simulink model "RLS_ADRC_2nd_order_Kang"  (R2024b)
settings: Solver=FixedStepAuto  StartTime=0.0  StopTime=250  FixedStep=T_sample  RelTol=1e-3
undefined symbols (not defined in the file): T_sample
settings Model: Creator=songk  LastModifiedBy=sk3547969879
settings RTWCC: GPUComputeCapability=3.5

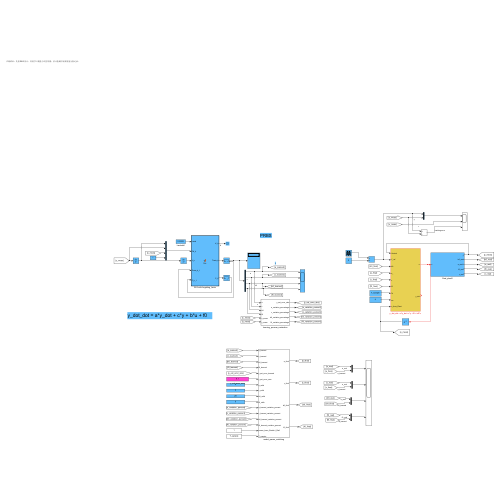
[thumbnail: Simulink's stored preview of the top-level diagram]
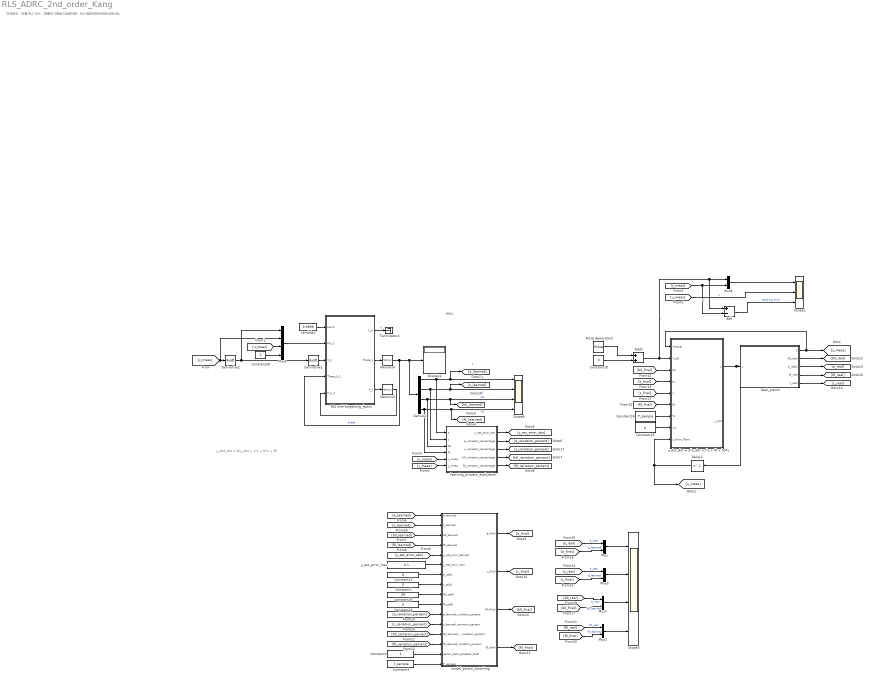
== system RLS_ADRC_2nd_order_Kang ==
  note: t
  note: PRBS
  note: y_dot_dot = a*y_dot + c*y + b*u + f0
  note: 在线辨识：先看 RLS 估计，再看学习使能与误差判据；估计值和控制采用值分别记录。
  Add : Sum  Inputs=+-
  Add2 : Sum
  Constant{1,20,22..23} (4 alike) : Constant  Value=0
  Constant2 : Constant
  Constant24 : Constant  Value=T_sample
  Constant25 : Constant  Value=4
  Constant26 : Constant  Value=28
  Constant28 : Constant
  Constant3 : Constant  Value=T_sample
  Delay2 : Delay  DelayLength=1
  Demux2 : Demux
  Derivative1 : Derivative
  Derivative2 : Derivative
  Display2 : Display
  Lambda2 : Constant  Value=0.9999
  Memory4 : Memory  InitialCondition=[1e-10;1e-10;1e-10;1e-10;]  InheritSampleTime=on
  Memory5 : Memory  InitialCondition=[1,0,0 0; 0,1,0 0; 0,0,1,0; 0 0 0 1]  InheritSampleTime=on
  Mux{,1..4} (5 alike) : Mux  Inputs=2
  Mux5 : Mux
  Pulse Generator2 : DiscretePulseGenerator  PulseType=Time based  Period=10  PulseWidth=50
  RLS with forgetting_factor : MATLAB Function  TreatAsAtomicUnit=on
  Real_plant2 : Subsystem
  Scope1 : Scope  NumInputPorts=3
  Scope3 : Scope  NumInputPorts=4
  Scope6 : Scope  NumInputPorts=4
  Terminator2 : Terminator
  learning_process_evaluation : Subsystem
  model_param_switching : Subsystem
  "y_dot_dot = a*y_dot +c*y + f0 + b0*u " : Subsystem
  y_est_error_max : Constant  Value=0.1
  wires:
  Real_plant2/1(y) -> "y_dot_dot = a*y_dot +c*y + f0 + b0*u "/1(Yactual), [y_meas]
  RLS with forgetting_factor/3(P_k) -> Memory5/1
  Derivative2/1 -> Derivative1/1, Mux5/1
  Memory4/1 -> RLS with forgetting_factor/4(Theta_k_1), Demux2/1, Display2/1  "theta"
  "y_dot_dot = a*y_dot +c*y + f0 + b0*u "/1(u) -> Delay2/1, Real_plant2/1(u)
  Mux4/1 -> Scope1/1
  RLS with forgetting_factor/2(Theta_k) -> Memory4/1
  Lambda2/1 -> RLS with forgetting_factor/1(Lamb)
  Demux2/4 -> Scope6/4, [f0_learned], learning_process_evaluation/4(f0)  "f0"
  Memory5/1 -> RLS with forgetting_factor/5(P_k_1)
  Pulse Generator2/1 -> Add2/1
  Constant28/1 -> Mux5/4
  Add2/1 -> Add/1, Mux4/1, "y_dot_dot = a*y_dot +c*y + f0 + b0*u "/2(Y_ref)  "r"
  Mux5/1 -> RLS with forgetting_factor/2(Phi_k)
  RLS with forgetting_factor/1(K_k) -> Terminator2/1  "K"
  Constant24/1 -> "y_dot_dot = a*y_dot +c*y + f0 + b0*u "/7(Ts)
  Constant20/1 -> Add2/2
  Constant25/1 -> "y_dot_dot = a*y_dot +c*y + f0 + b0*u "/8(wc)
  [y_meas] -> Mux5/2, Derivative2/1
  [u_meas] -> Mux5/3
  [y_meas] -> Add/2, Mux4/2  "y"
  [u_meas] -> Scope1/2  "u"
  Demux2/1 -> [a_learned], Scope6/1, learning_process_evaluation/1(a)  "a"
  Demux2/3 -> Scope6/3, [b0_learned], learning_process_evaluation/3(b0)  "b0"
  learning_process_evaluation/2(a_variation_percentage) -> [a_variation_percent]
  learning_process_evaluation/1(y_est_error_abs) -> [y_est_error_abs]
  learning_process_evaluation/4(b0_variation_percentage) -> [b0_variation_percent]
  learning_process_evaluation/5(f0_variation_percentage) -> [f0_variation_percent]
  [y_meas] -> learning_process_evaluation/6(y_meas)
  [u_meas] -> learning_process_evaluation/5(u_meas)
  [a_learned] -> model_param_switching/1(a_learned)
  [b0_learned] -> model_param_switching/3(b0_learned)
  [f0_learned] -> model_param_switching/4(f0_learned)
  [y_est_error_abs] -> model_param_switching/5(y_est_error_learned)
  y_est_error_max/1 -> model_param_switching/6(y_est_erorr_max)
  Constant23/1 -> model_param_switching/7(a_calib)
  Constant26/1 -> model_param_switching/9(b0_calib)
  Constant22/1 -> model_param_switching/10(f0_calib)
  [a_variation_percent] -> model_param_switching/11(a_learned_variation_percent)
  [b0_variation_percent] -> model_param_switching/13(b0_learned_variation_percent)
  model_param_switching/1(a_final) -> [a_final]
  model_param_switching/3(b0_final) -> [b0_final]
  [a_final] -> "y_dot_dot = a*y_dot +c*y + f0 + b0*u "/4(a_)
  [b0_final] -> "y_dot_dot = a*y_dot +c*y + f0 + b0*u "/3(b0)
  [f0_final] -> "y_dot_dot = a*y_dot +c*y + f0 + b0*u "/6(f0)
  Real_plant2/2(b0_real) -> [b0_real]
  Real_plant2/3(a_real1) -> [a_real]
  Real_plant2/5(c_real) -> [c_real]
  [a_real] -> Mux/1  "a_real"
  [a_final] -> Mux/2  "a_learned"
  [b0_real] -> Mux1/1  "b_real"
  [b0_final] -> Mux1/2  "b0_learned"
  [f0_real] -> Mux2/1  "f0_real"
  [f0_final] -> Mux2/2  "f0_learned"
  Mux/1 -> Scope3/1
  Mux1/1 -> Scope3/3
  Mux2/1 -> Scope3/4
  Add/1 -> Scope1/3  "tracking error"
  Real_plant2/4(f0_real) -> [f0_real]
  [c_final] -> "y_dot_dot = a*y_dot +c*y + f0 + b0*u "/5(c)
  Mux3/1 -> Scope3/2
  [c_final] -> Mux3/2  "a_learned"
  [c_real] -> Mux3/1  "a_real"
  model_param_switching/2(c_final) -> [c_final]
  model_param_switching/4(f0_final) -> [f0_final]
  Constant3/1 -> model_param_switching/16(T_sample)
  [f0_variation_percent] -> model_param_switching/14(f0_learned_variation_percent)
  [c_variation_percent] -> model_param_switching/12(c_learned_variation_percent)
  Constant1/1 -> model_param_switching/8(c_calib)
  [c_learned] -> model_param_switching/2(c_learned)
  learning_process_evaluation/3(c_variation_percentage) -> [c_variation_percent]
  Demux2/2 -> learning_process_evaluation/2(c), [c_learned], Scope6/2  "c"
  Derivative1/1 -> RLS with forgetting_factor/3(Y_k)
  Constant2/1 -> model_param_switching/15(param_learn_Enable1_Dis0)
  Delay2/1 -> "y_dot_dot = a*y_dot +c*y + f0 + b0*u "/9(u_from_Plant), [u_meas]

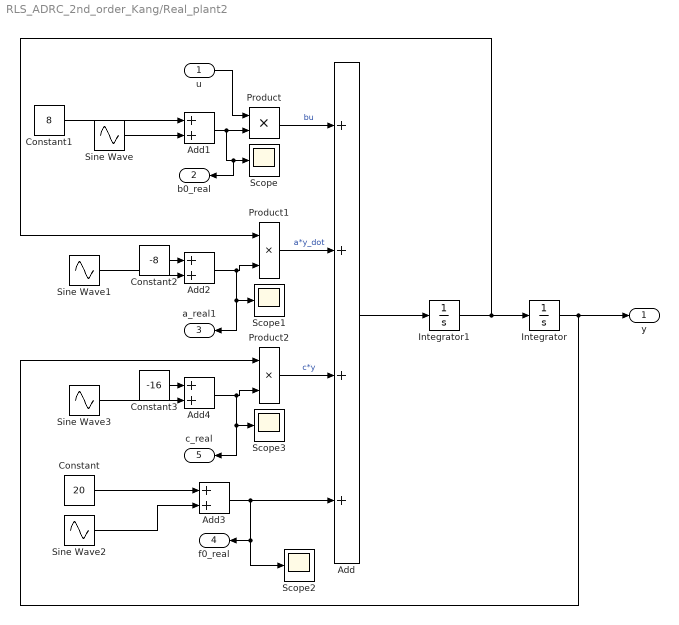
== system RLS_ADRC_2nd_order_Kang/Real_plant2 ==
  u : Inport
  Add : Sum  Inputs=++++
  Add{1..4} (4 alike) : Sum
  Constant : Constant  Value=20
  Constant1 : Constant  Value=8
  Constant2 : Constant  Value=-8
  Constant3 : Constant  Value=-16
  Integrator : Integrator
  Integrator1 : Integrator
  Product : Product
  Product1 : Product
  Product2 : Product
  Scope{,1..3} (4 alike) : Scope
  Sine Wave : Sin  Amplitude=10*0  Frequency=0.0125*2  SampleTime=0
  Sine Wave1 : Sin  Amplitude=0.2*0  Frequency=0.0125*2  Phase=90/180*pi  SampleTime=0
  Sine Wave2 : Sin  Amplitude=100*0  Frequency=0.009*3  Phase=180/180*pi  SampleTime=0
  Sine Wave3 : Sin  Amplitude=0.2*0  Frequency=0.0125*2  Phase=90/180*pi  SampleTime=0
  y : Outport
  b0_real : Outport  Port=2
  a_real1 : Outport  Port=3
  f0_real : Outport  Port=4
  c_real : Outport  Port=5
  wires:
  Add/1 -> Integrator1/1
  u/1 -> Product/1
  Constant1/1 -> Add1/1
  Constant2/1 -> Add2/1
  Constant/1 -> Add3/1
  Sine Wave/1 -> Add1/2
  Sine Wave1/1 -> Add2/2
  Sine Wave2/1 -> Add3/2
  Add2/1 -> a_real1/1, Scope1/1, Product1/2
  Add1/1 -> b0_real/1, Scope/1, Product/2
  Product/1 -> Add/1  "bu"
  Product1/1 -> Add/2  "a*y_dot"
  Integrator1/1 -> Product1/1, Integrator/1
  Add3/1 -> Scope2/1, f0_real/1, Add/4
  Integrator/1 -> Product2/1, y/1
  Add4/1 -> Product2/2, Scope3/1, c_real/1
  Sine Wave3/1 -> Add4/2
  Constant3/1 -> Add4/1
  Product2/1 -> Add/3  "c*y"

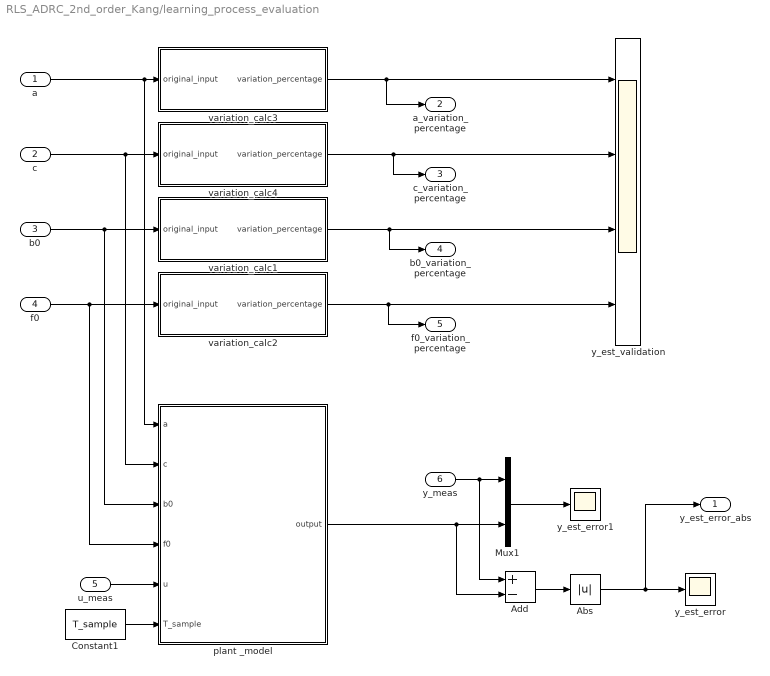
== system RLS_ADRC_2nd_order_Kang/learning_process_evaluation ==
  a : Inport
  c : Inport  Port=2
  b0 : Inport  Port=3
  f0 : Inport  Port=4
  u_meas : Inport  Port=5
  y_meas : Inport  Port=6
  Abs : Abs  SaturateOnIntegerOverflow=off
  Add : Sum  Inputs=+-
  Constant1 : Constant  Value=T_sample
  Mux1 : Mux  Inputs=2
  plant _model : Subsystem
  variation_calc1 : Subsystem
  variation_calc2 : Subsystem
  variation_calc3 : Subsystem
  variation_calc4 : Subsystem
  y_est_error : Scope
  y_est_error1 : Scope
  y_est_validation : Scope  NumInputPorts=4
  y_est_error_abs : Outport
  a_variation_percentage : Outport  Port=2
  c_variation_percentage : Outport  Port=3
  b0_variation_percentage : Outport  Port=4
  f0_variation_percentage : Outport  Port=5
  wires:
  b0/1 -> variation_calc1/1(original_input), plant _model/3(b0)
  y_meas/1 -> Add/1, Mux1/1
  Constant1/1 -> plant _model/6(T_sample)
  Add/1 -> Abs/1
  Abs/1 -> y_est_error_abs/1, y_est_error/1
  Mux1/1 -> y_est_error1/1
  variation_calc2/1(variation_percentage) -> y_est_validation/4, f0_variation_percentage/1
  plant _model/1(output) -> Add/2, Mux1/2
  a/1 -> variation_calc3/1(original_input), plant _model/1(a)
  variation_calc3/1(variation_percentage) -> a_variation_percentage/1, y_est_validation/1
  variation_calc1/1(variation_percentage) -> y_est_validation/3, b0_variation_percentage/1
  f0/1 -> plant _model/4(f0), variation_calc2/1(original_input)
  u_meas/1 -> plant _model/5(u)
  variation_calc4/1(variation_percentage) -> c_variation_percentage/1, y_est_validation/2
  c/1 -> plant _model/2(c), variation_calc4/1(original_input)

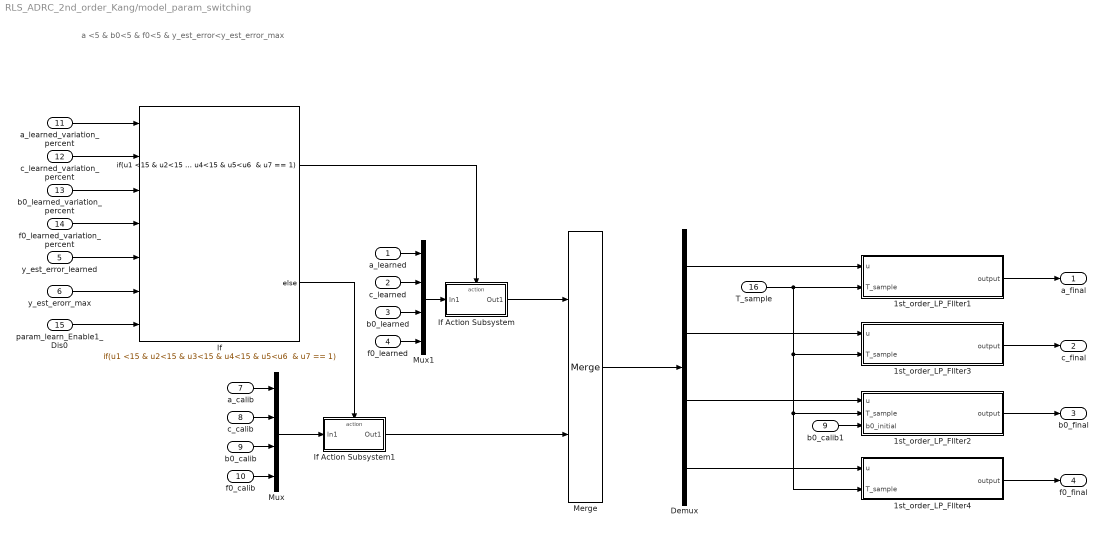
== system RLS_ADRC_2nd_order_Kang/model_param_switching ==
  note: a <5 & b0<5 & f0<5 & y_est_error<y_est_error_max
  a_learned : Inport
  c_learned : Inport  Port=2
  b0_learned : Inport  Port=3
  f0_learned : Inport  Port=4
  y_est_error_learned : Inport  Port=5
  y_est_erorr_max : Inport  Port=6
  a_calib : Inport  Port=7
  c_calib : Inport  Port=8
  b0_calib : Inport  Port=9
  f0_calib : Inport  Port=10
  a_learned_variation_percent : Inport  Port=11
  c_learned_variation_percent : Inport  Port=12
  b0_learned_variation_percent : Inport  Port=13
  f0_learned_variation_percent : Inport  Port=14
  param_learn_Enable1_Dis0 : Inport  Port=15
  T_sample : Inport  Port=16
  1st_order_LP_FIlter1 : Subsystem
  1st_order_LP_FIlter2 : Subsystem
  1st_order_LP_FIlter3 : Subsystem
  1st_order_LP_FIlter4 : Subsystem
  Demux : Demux
  If : If  NumInputs=7  IfExpression="u1 <15 & u2<15 & u3<15 & u4<15 & u5<u6  & u7 == 1"
  If Action Subsystem : Subsystem  TreatAsAtomicUnit=on
  If Action Subsystem1 : Subsystem  TreatAsAtomicUnit=on
  Merge : Merge
  Mux : Mux
  Mux1 : Mux
  b0_calib1 : InportShadow  Port=9
  a_final : Outport
  c_final : Outport  Port=2
  b0_final : Outport  Port=3
  f0_final : Outport  Port=4
  wires:
  Mux/1 -> If Action Subsystem1/1(In1)
  If Action Subsystem/1(Out1) -> Merge/1
  If/2 -> If Action Subsystem1/Action
  If Action Subsystem1/1(Out1) -> Merge/2
  If/1 -> If Action Subsystem/Action
  a_calib/1 -> Mux/1
  b0_calib/1 -> Mux/3
  f0_calib/1 -> Mux/4
  Mux1/1 -> If Action Subsystem/1(In1)
  a_learned/1 -> Mux1/1
  a_learned_variation_percent/1 -> If/1
  Merge/1 -> Demux/1
  Demux/3 -> 1st_order_LP_FIlter2/1(u)
  Demux/1 -> 1st_order_LP_FIlter1/1(u)
  1st_order_LP_FIlter1/1(output) -> a_final/1
  1st_order_LP_FIlter2/1(output) -> b0_final/1
  1st_order_LP_FIlter3/1(output) -> c_final/1
  b0_calib1/1 -> 1st_order_LP_FIlter2/3(b0_initial)
  1st_order_LP_FIlter4/1(output) -> f0_final/1
  Demux/2 -> 1st_order_LP_FIlter3/1(u)
  T_sample/1 -> 1st_order_LP_FIlter1/2(T_sample), 1st_order_LP_FIlter4/2(T_sample), 1st_order_LP_FIlter2/2(T_sample), 1st_order_LP_FIlter3/2(T_sample)
  Demux/4 -> 1st_order_LP_FIlter4/1(u)
  c_calib/1 -> Mux/2
  c_learned/1 -> Mux1/2
  b0_learned/1 -> Mux1/3
  f0_learned/1 -> Mux1/4
  c_learned_variation_percent/1 -> If/2
  b0_learned_variation_percent/1 -> If/3
  f0_learned_variation_percent/1 -> If/4
  y_est_error_learned/1 -> If/5
  y_est_erorr_max/1 -> If/6
  param_learn_Enable1_Dis0/1 -> If/7

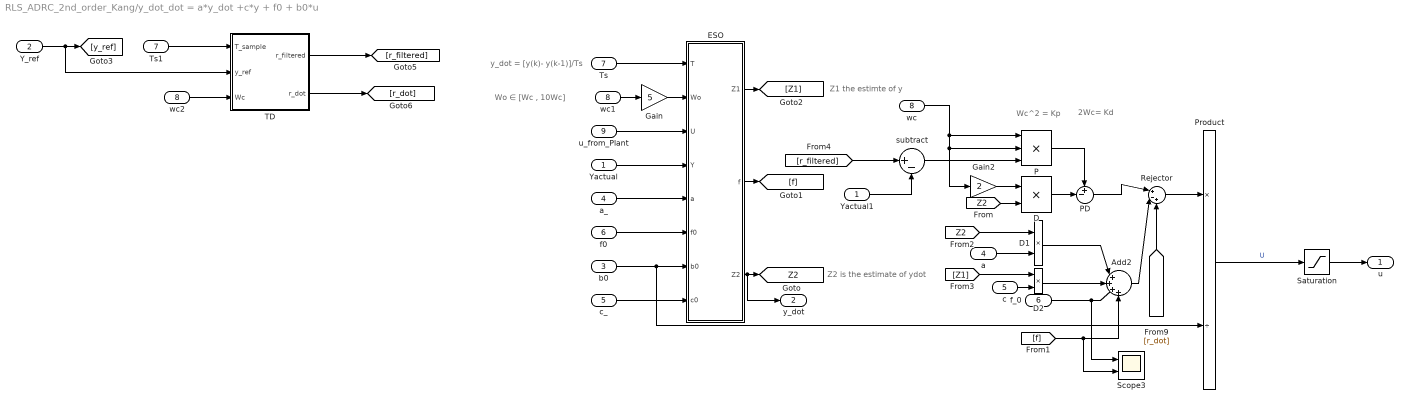
== system RLS_ADRC_2nd_order_Kang/y_dot_dot = a*y_dot +c*y + f0 + b0*u  ==
  note: 2Wc= Kd
  note: Wc^2 = Kp
  note: Z2 is the estimate of ydot
  note: Z1 the estimte of y
  note: Wo ∈ [Wc , 10Wc]
  note: y_dot = [y(k)- y(k-1)]/Ts
  Yactual : Inport
  Y_ref : Inport  Port=2
  b0 : Inport  Port=3
  a_ : Inport  Port=4
  c : Inport  Port=5
  f0 : Inport  Port=6
  Ts : Inport  Port=7
  wc : Inport  Port=8
  u_from_Plant : Inport  Port=9
  Add2 : Sum  Inputs=|++++
  D : Product  RndMeth=Zero
  D1 : Product  RndMeth=Zero
  D2 : Product  RndMeth=Zero
  ESO : Subsystem
  Gain : Gain  Gain=5
  Gain2 : Gain  Gain=2
  P : Product  Inputs=3  RndMeth=Zero
  PD : Sum  Inputs=+-|
  Product : Product  Inputs=*/  RndMeth=Zero
  Rejector : Sum  Inputs=|+-+
  Saturation : Saturate  UpperLimit=inf  LowerLimit=-inf
  Scope3 : Scope  NumInputPorts=2
  TD : Subsystem
  Ts1 : InportShadow  Port=7
  Yactual1 : InportShadow
  a : InportShadow  Port=4
  c_ : InportShadow  Port=5
  f_0 : InportShadow  Port=6
  subtract : Sum  Inputs=|+-
  wc1 : InportShadow  Port=8
  wc2 : InportShadow  Port=8
  u : Outport  VectorParamsAs1DForOutWhenUnconnected=off
  y_dot : Outport  Port=2  VectorParamsAs1DForOutWhenUnconnected=off
  tag scope: Z2=global
  wires:
  [Z2] -> D1/1
  a/1 -> D1/2
  D1/1 -> Add2/1
  Ts/1 -> ESO/1(T)
  wc1/1 -> Gain/1
  u_from_Plant/1 -> ESO/3(U)
  Yactual/1 -> ESO/4(Y)
  a_/1 -> ESO/5(a)
  f0/1 -> ESO/6(f0)
  ESO/2(f) -> [f]
  [Z2] -> D/2
  b0/1 -> Product/2, ESO/7(b0)
  Product/1 -> Saturation/1  "U"
  subtract/1 -> P/3
  Gain2/1 -> D/1
  wc/1 -> Gain2/1, P/2, P/1
  P/1 -> PD/1
  ESO/3(Z2) -> y_dot/1, [Z2]
  D/1 -> PD/2
  PD/1 -> Rejector/1
  f_0/1 -> Scope3/1, Add2/3
  [f] -> Scope3/2, Add2/4
  Add2/1 -> Rejector/2
  Rejector/1 -> Product/1
  c_/1 -> ESO/8(c0)
  c/1 -> D2/2
  Yactual1/1 -> subtract/2
  D2/1 -> Add2/2
  ESO/1(Z1) -> [Z1]
  [Z1] -> D2/1
  Gain/1 -> ESO/2(Wo)
  [r_dot] -> Rejector/3
  Saturation/1 -> u/1
  [r_filtered] -> subtract/1
  Ts1/1 -> TD/1(T_sample)
  Y_ref/1 -> TD/2(y_ref), [y_ref]
  TD/1(r_filtered) -> [r_filtered]
  TD/2(r_dot) -> [r_dot]
  wc2/1 -> TD/3(Wc)

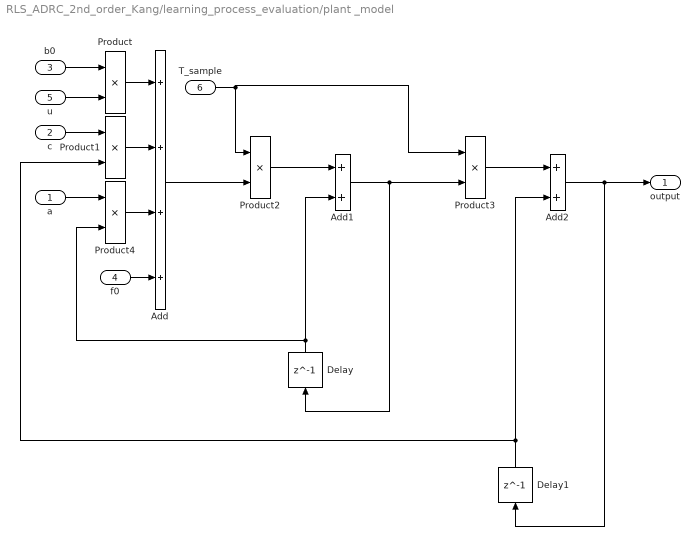
== system RLS_ADRC_2nd_order_Kang/learning_process_evaluation/plant _model ==
  a : Inport
  c : Inport  Port=2
  b0 : Inport  Port=3
  f0 : Inport  Port=4
  u : Inport  Port=5
  T_sample : Inport  Port=6
  Add : Sum  Inputs=++++
  Add1 : Sum
  Add2 : Sum
  Delay : Delay  DelayLength=1
  Delay1 : Delay  DelayLength=1
  Product{,1..4} (5 alike) : Product
  output : Outport
  wires:
  Add/1 -> Product2/2
  u/1 -> Product/2
  Product/1 -> Add/1
  a/1 -> Product4/1
  f0/1 -> Add/4
  b0/1 -> Product/1
  Product1/1 -> Add/2
  T_sample/1 -> Product2/1, Product3/1
  Product2/1 -> Add1/1
  Add1/1 -> Product3/2, Delay/1
  Delay/1 -> Product4/2, Add1/2
  Delay1/1 -> Product1/2, Add2/2
  Add2/1 -> output/1, Delay1/1
  Product3/1 -> Add2/1
  Product4/1 -> Add/3
  c/1 -> Product1/1

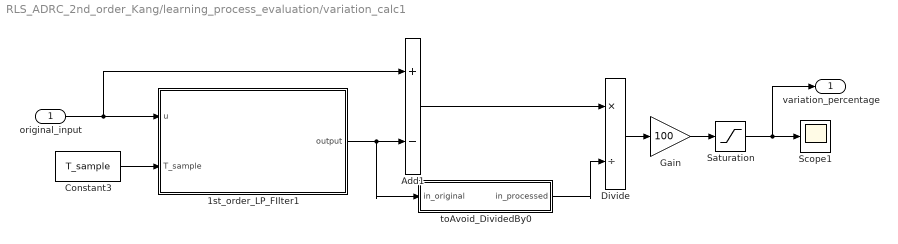
== system RLS_ADRC_2nd_order_Kang/learning_process_evaluation/variation_calc1 ==
  original_input : Inport
  1st_order_LP_FIlter1 : Subsystem
  Add1 : Sum  Inputs=+-
  Constant3 : Constant  Value=T_sample
  Divide : Product  Inputs=*/
  Gain : Gain  Gain=100
  Saturation : Saturate  UpperLimit=100  LowerLimit=-100
  Scope1 : Scope
  toAvoid_DividedBy0 : Subsystem
  variation_percentage : Outport
  wires:
  Divide/1 -> Gain/1
  1st_order_LP_FIlter1/1(output) -> Add1/2, toAvoid_DividedBy0/1(in_original)
  toAvoid_DividedBy0/1(in_processed) -> Divide/2
  original_input/1 -> 1st_order_LP_FIlter1/1(u), Add1/1
  Constant3/1 -> 1st_order_LP_FIlter1/2(T_sample)
  Add1/1 -> Divide/1
  Gain/1 -> Saturation/1
  Saturation/1 -> Scope1/1, variation_percentage/1

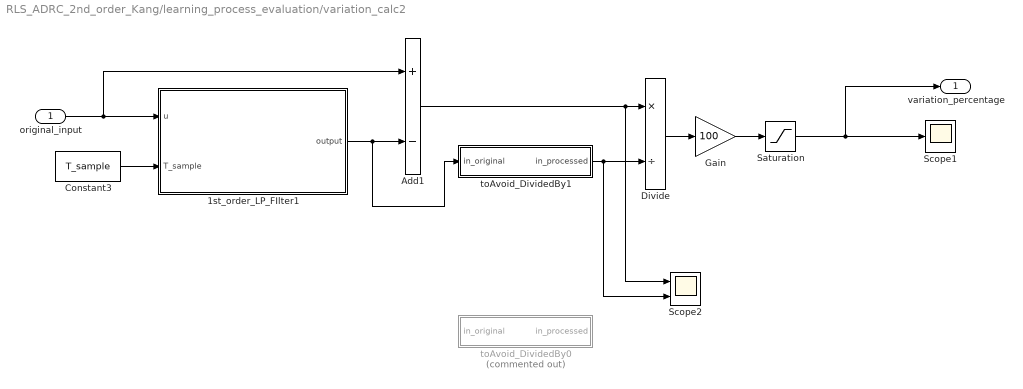
== system RLS_ADRC_2nd_order_Kang/learning_process_evaluation/variation_calc2 ==
  original_input : Inport
  1st_order_LP_FIlter1 : Subsystem
  Add1 : Sum  Inputs=+-
  Constant3 : Constant  Value=T_sample
  Divide : Product  Inputs=*/
  Gain : Gain  Gain=100
  Saturation : Saturate  UpperLimit=100  LowerLimit=-100
  Scope1 : Scope
  Scope2 : Scope  NumInputPorts=2
  toAvoid_DividedBy0 : Subsystem  Commented=on
  toAvoid_DividedBy1 : Subsystem
  variation_percentage : Outport
  wires:
  Gain/1 -> Saturation/1
  Add1/1 -> Scope2/1, Divide/1
  Constant3/1 -> 1st_order_LP_FIlter1/2(T_sample)
  original_input/1 -> Add1/1, 1st_order_LP_FIlter1/1(u)
  toAvoid_DividedBy1/1(in_processed) -> Scope2/2, Divide/2
  1st_order_LP_FIlter1/1(output) -> toAvoid_DividedBy1/1(in_original), Add1/2
  Divide/1 -> Gain/1
  Saturation/1 -> variation_percentage/1, Scope1/1

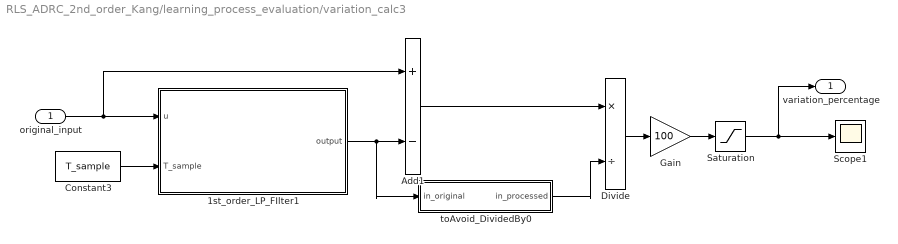
== system RLS_ADRC_2nd_order_Kang/learning_process_evaluation/variation_calc3 ==
  original_input : Inport
  1st_order_LP_FIlter1 : Subsystem
  Add1 : Sum  Inputs=+-
  Constant3 : Constant  Value=T_sample
  Divide : Product  Inputs=*/
  Gain : Gain  Gain=100
  Saturation : Saturate  UpperLimit=100  LowerLimit=-100
  Scope1 : Scope
  toAvoid_DividedBy0 : Subsystem
  variation_percentage : Outport
  wires:
  Gain/1 -> Saturation/1
  Add1/1 -> Divide/1
  Constant3/1 -> 1st_order_LP_FIlter1/2(T_sample)
  original_input/1 -> Add1/1, 1st_order_LP_FIlter1/1(u)
  toAvoid_DividedBy0/1(in_processed) -> Divide/2
  1st_order_LP_FIlter1/1(output) -> toAvoid_DividedBy0/1(in_original), Add1/2
  Divide/1 -> Gain/1
  Saturation/1 -> variation_percentage/1, Scope1/1

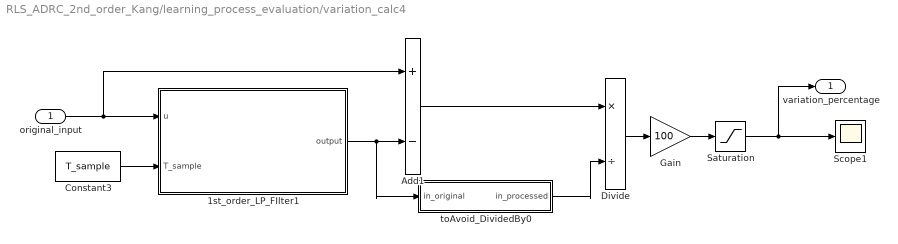
== system RLS_ADRC_2nd_order_Kang/learning_process_evaluation/variation_calc4 ==
  original_input : Inport
  1st_order_LP_FIlter1 : Subsystem
  Add1 : Sum  Inputs=+-
  Constant3 : Constant  Value=T_sample
  Divide : Product  Inputs=*/
  Gain : Gain  Gain=100
  Saturation : Saturate  UpperLimit=100  LowerLimit=-100
  Scope1 : Scope
  toAvoid_DividedBy0 : Subsystem
  variation_percentage : Outport
  wires:
  Saturation/1 -> Scope1/1, variation_percentage/1
  Divide/1 -> Gain/1
  1st_order_LP_FIlter1/1(output) -> Add1/2, toAvoid_DividedBy0/1(in_original)
  toAvoid_DividedBy0/1(in_processed) -> Divide/2
  original_input/1 -> 1st_order_LP_FIlter1/1(u), Add1/1
  Constant3/1 -> 1st_order_LP_FIlter1/2(T_sample)
  Add1/1 -> Divide/1
  Gain/1 -> Saturation/1

== system RLS_ADRC_2nd_order_Kang/model_param_switching/1st_order_LP_FIlter1 ==
  u : Inport
  T_sample : Inport  Port=2
  Add : Sum  Inputs=+-
  Add1 : Sum
  Delay : Delay  DelayLength=1
  Divide : Product  Inputs=*/
  Product2 : Product
  "tau_LPF " : Constant  Value=3
  output : Outport
  wires:
  Add/1 -> Product2/2
  u/1 -> Add/1
  Add1/1 -> Delay/1, output/1
  T_sample/1 -> Product2/1
  Product2/1 -> Divide/1
  Delay/1 -> Add/2, Add1/2
  Divide/1 -> Add1/1
  "tau_LPF "/1 -> Divide/2

== system RLS_ADRC_2nd_order_Kang/model_param_switching/1st_order_LP_FIlter2 ==
  u : Inport
  T_sample : Inport  Port=2
  b0_initial : Inport  Port=3
  Add : Sum  Inputs=+-
  Add1 : Sum
  Delay : Delay  DelayLength=1  InitialConditionSource=Input port  InitialCondition=-100
      settings: InputPortMap=u0,p4
  Divide : Product  Inputs=*/
  Product2 : Product
  "tau_LPF " : Constant  Value=3
  output : Outport
  wires:
  "tau_LPF "/1 -> Divide/2
  Divide/1 -> Add1/1
  Delay/1 -> Add1/2, Add/2
  Product2/1 -> Divide/1
  T_sample/1 -> Product2/1
  Add1/1 -> output/1, Delay/1
  u/1 -> Add/1
  Add/1 -> Product2/2
  b0_initial/1 -> Delay/2

== system RLS_ADRC_2nd_order_Kang/model_param_switching/1st_order_LP_FIlter3 ==
  u : Inport
  T_sample : Inport  Port=2
  Add : Sum  Inputs=+-
  Add1 : Sum
  Delay : Delay  DelayLength=1
  Divide : Product  Inputs=*/
  Product2 : Product
  "tau_LPF " : Constant  Value=3
  output : Outport
  wires:
  Add/1 -> Product2/2
  u/1 -> Add/1
  Add1/1 -> Delay/1, output/1
  T_sample/1 -> Product2/1
  Product2/1 -> Divide/1
  Delay/1 -> Add/2, Add1/2
  Divide/1 -> Add1/1
  "tau_LPF "/1 -> Divide/2

== system RLS_ADRC_2nd_order_Kang/model_param_switching/1st_order_LP_FIlter4 ==
  u : Inport
  T_sample : Inport  Port=2
  Add : Sum  Inputs=+-
  Add1 : Sum
  Delay : Delay  DelayLength=1
  Divide : Product  Inputs=*/
  Product2 : Product
  "tau_LPF " : Constant  Value=3
  output : Outport
  wires:
  "tau_LPF "/1 -> Divide/2
  Divide/1 -> Add1/1
  Delay/1 -> Add1/2, Add/2
  Product2/1 -> Divide/1
  T_sample/1 -> Product2/1
  Add1/1 -> output/1, Delay/1
  u/1 -> Add/1
  Add/1 -> Product2/2

== system RLS_ADRC_2nd_order_Kang/model_param_switching/If Action Subsystem ==
  In1 : Inport
  Action Port : ActionPort  ActionPortLabel="if(u1 <15 & u2<15 & u3<15 & u4<15 & u5<u6  & u7 == 1)"
  Out1 : Outport
  wires:
  In1/1 -> Out1/1

== system RLS_ADRC_2nd_order_Kang/model_param_switching/If Action Subsystem1 ==
  In1 : Inport
  Action Port : ActionPort  ActionPortLabel=else
  Out1 : Outport
  wires:
  In1/1 -> Out1/1

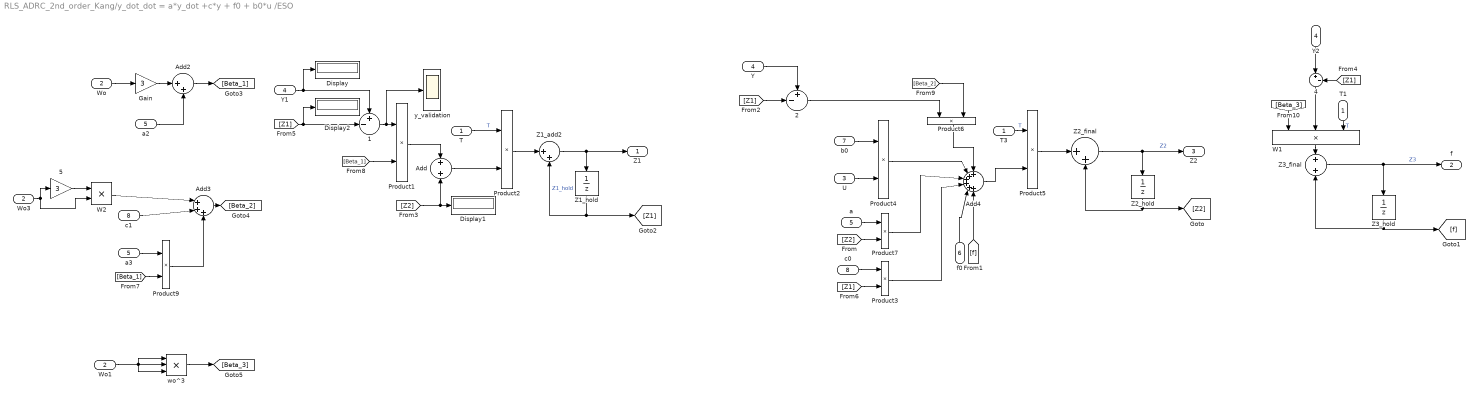
== system RLS_ADRC_2nd_order_Kang/y_dot_dot = a*y_dot +c*y + f0 + b0*u /ESO ==
  T : Inport
  Wo : Inport  Port=2
  U : Inport  Port=3
  Y : Inport  Port=4
  a : Inport  Port=5
  f0 : Inport  Port=6
  b0 : Inport  Port=7
  c0 : Inport  Port=8
  1 : Sum  Inputs=+-|
  2 : Sum  Inputs=+-|
  4 : Sum  Inputs=|+-
  5 : Gain  Gain=3
  Add : Sum
  Add2 : Sum  Inputs=|++
  Add3 : Sum  Inputs=|+++
  Add4 : Sum  Inputs=++++++
  Display : Display
  Display1 : Display
  Display2 : Display
  Gain : Gain  Gain=3
  Product{1..7,9} (8 alike) : Product  RndMeth=Zero
  T1 : InportShadow
  T3 : InportShadow
  W1 : Product  Inputs=3  RndMeth=Zero
  W2 : Product  RndMeth=Zero
  Wo1 : InportShadow  Port=2
  Wo3 : InportShadow  Port=2
  Y1 : InportShadow  Port=4
  Y2 : InportShadow  Port=4
  Z1_add2 : Sum  Inputs=|++
  Z1_hold : UnitDelay  SampleTime=-1  HasFrameUpgradeWarning=on
  Z2_final : Sum  Inputs=|++
  Z2_hold : UnitDelay  SampleTime=-1  HasFrameUpgradeWarning=on
  Z3_final : Sum
  Z3_hold : UnitDelay  SampleTime=-1  HasFrameUpgradeWarning=on
  a2 : InportShadow  Port=5
  a3 : InportShadow  Port=5
  c1 : InportShadow  Port=8
  wo^3 : Product  Inputs=3  RndMeth=Zero
  y_validation : Scope
  Z1 : Outport  VectorParamsAs1DForOutWhenUnconnected=off
  f : Outport  Port=2  VectorParamsAs1DForOutWhenUnconnected=off
  Z2 : Outport  Port=3  VectorParamsAs1DForOutWhenUnconnected=off
  wires:
  Z3_hold/1 -> [f], Z3_final/2
  f0/1 -> Add4/5
  Y1/1 -> Display/1, 1/1
  [Z1] -> Display2/1, 1/2
  Wo1/1 -> wo^3/1, wo^3/2, wo^3/3
  [Z1] -> 4/2
  Y2/1 -> 4/1
  4/1 -> W1/2
  [Z2] -> Add/2, Display1/1
  Y/1 -> 2/1
  [Z1] -> 2/2
  [Z2] -> Product7/2
  T3/1 -> Product5/1  "T"
  T1/1 -> W1/3  "T"
  Product7/1 -> Add4/3
  a/1 -> Product7/1
  Product6/1 -> Add4/1
  [Beta_1] -> Product1/2
  1/1 -> y_validation/1, Product1/1
  Product1/1 -> Add/1
  T/1 -> Product2/1  "T"
  Add/1 -> Product2/2
  Product2/1 -> Z1_add2/1
  Z1_add2/1 -> Z1_hold/1, Z1/1
  Product4/1 -> Add4/2
  2/1 -> Product6/1
  Add4/1 -> Product5/2
  Product5/1 -> Z2_final/1
  [Beta_3] -> W1/1
  W1/1 -> Z3_final/1
  Z2_final/1 -> Z2/1, Z2_hold/1  "Z2"
  U/1 -> Product4/2
  Z1_hold/1 -> Z1_add2/2, [Z1]  "Z1_hold"
  Z2_hold/1 -> [Z2], Z2_final/2
  Z3_final/1 -> Z3_hold/1, f/1  "Z3"
  b0/1 -> Product4/1
  Wo/1 -> Gain/1
  Product3/1 -> Add4/4
  [Z1] -> Product3/2
  c0/1 -> Product3/1
  wo^3/1 -> [Beta_3]
  Gain/1 -> Add2/1
  Add2/1 -> [Beta_1]
  a2/1 -> Add2/2
  Wo3/1 -> 5/1, W2/2
  5/1 -> W2/1
  W2/1 -> Add3/1
  c1/1 -> Add3/2
  a3/1 -> Product9/1
  Add3/1 -> [Beta_2]
  [Beta_1] -> Product9/2
  Product9/1 -> Add3/3
  [Beta_2] -> Product6/2
  [f] -> Add4/6

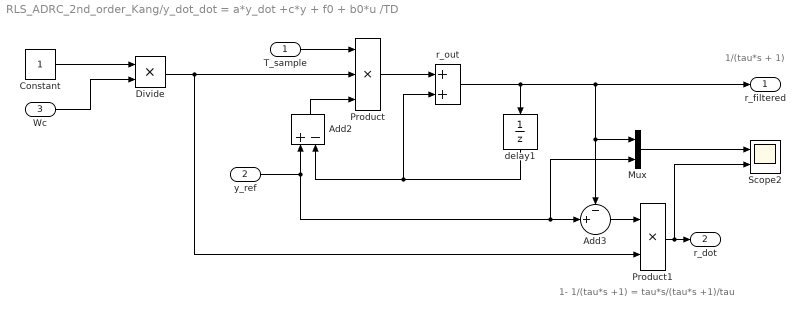
== system RLS_ADRC_2nd_order_Kang/y_dot_dot = a*y_dot +c*y + f0 + b0*u /TD ==
  note: 1- 1/(tau*s +1) = tau*s/(tau*s +1)/tau
  note: 1/(tau*s + 1)
  T_sample : Inport
  y_ref : Inport  Port=2
  Wc : Inport  Port=3
  Add2 : Sum  Inputs=+-
  Add3 : Sum  Inputs=-+|
  Constant : Constant
  Divide : Product  Inputs=**
  Mux : Mux  Inputs=2
  Product : Product  Inputs=3  RndMeth=Zero
  Product1 : Product  RndMeth=Zero
  Scope2 : Scope  NumInputPorts=2
  delay1 : UnitDelay  SampleTime=-1  HasFrameUpgradeWarning=on
  r_out : Sum
  r_filtered : Outport  VectorParamsAs1DForOutWhenUnconnected=off
  r_dot : Outport  Port=2  VectorParamsAs1DForOutWhenUnconnected=off
  wires:
  T_sample/1 -> Product/1
  Divide/1 -> Product/2, Product1/2
  Add3/1 -> Product1/1
  r_out/1 -> r_filtered/1, Mux/1, Add3/1, delay1/1
  Add2/1 -> Product/3
  Product1/1 -> Scope2/2, r_dot/1
  delay1/1 -> r_out/2, Add2/2
  y_ref/1 -> Mux/2, Add3/2, Add2/1
  Product/1 -> r_out/1
  Mux/1 -> Scope2/1
  Constant/1 -> Divide/1
  Wc/1 -> Divide/2

== system RLS_ADRC_2nd_order_Kang/learning_process_evaluation/variation_calc1/1st_order_LP_FIlter1 ==
  u : Inport
  T_sample : Inport  Port=2
  Add : Sum  Inputs=+-
  Add1 : Sum
  Delay : Delay  DelayLength=1
  Divide : Product  Inputs=*/
  Product2 : Product
  "tau_LPF " : Constant
  output : Outport
  wires:
  "tau_LPF "/1 -> Divide/2
  Divide/1 -> Add1/1
  Delay/1 -> Add1/2, Add/2
  Product2/1 -> Divide/1
  T_sample/1 -> Product2/1
  Add1/1 -> output/1, Delay/1
  u/1 -> Add/1
  Add/1 -> Product2/2

== system RLS_ADRC_2nd_order_Kang/learning_process_evaluation/variation_calc1/toAvoid_DividedBy0 ==
  in_original : Inport
  Add3 : Sum
  Constant : Constant  Value=1e-10
  If : If  IfExpression=u1 == 0
  If Action Subsystem : Subsystem  TreatAsAtomicUnit=on
  If Action Subsystem1 : Subsystem  TreatAsAtomicUnit=on
  Merge : Merge
  in_processed : Outport
  wires:
  Merge/1 -> in_processed/1
  If/1 -> If Action Subsystem/Action
  If Action Subsystem1/1(Out1) -> Merge/2
  If/2 -> If Action Subsystem1/Action
  Constant/1 -> Add3/2
  If Action Subsystem/1(Out1) -> Merge/1
  Add3/1 -> If Action Subsystem1/1(In1)
  in_original/1 -> If/1, If Action Subsystem/1(In1), Add3/1

== system RLS_ADRC_2nd_order_Kang/learning_process_evaluation/variation_calc2/1st_order_LP_FIlter1 ==
  u : Inport
  T_sample : Inport  Port=2
  Add : Sum  Inputs=+-
  Add1 : Sum
  Delay : Delay  DelayLength=1
  Divide : Product  Inputs=*/
  Product2 : Product
  "tau_LPF " : Constant
  output : Outport
  wires:
  Add/1 -> Product2/2
  u/1 -> Add/1
  Add1/1 -> Delay/1, output/1
  T_sample/1 -> Product2/1
  Product2/1 -> Divide/1
  Delay/1 -> Add/2, Add1/2
  Divide/1 -> Add1/1
  "tau_LPF "/1 -> Divide/2

== system RLS_ADRC_2nd_order_Kang/learning_process_evaluation/variation_calc2/toAvoid_DividedBy0 ==
  in_original : Inport
  Constant : Constant  Value=1e-1
  If : If  IfExpression=u1 < 1e-1 | u1>-1e-1
  If Action Subsystem : Subsystem  TreatAsAtomicUnit=on
  If Action Subsystem1 : Subsystem  TreatAsAtomicUnit=on
  Merge : Merge
  in_processed : Outport
  wires:
  If Action Subsystem/1(Out1) -> Merge/1
  If/2 -> If Action Subsystem1/Action
  If Action Subsystem1/1(Out1) -> Merge/2
  If/1 -> If Action Subsystem/Action
  Merge/1 -> in_processed/1
  Constant/1 -> If Action Subsystem/1(In1)
  in_original/1 -> If Action Subsystem1/1(in_original), If/1

== system RLS_ADRC_2nd_order_Kang/learning_process_evaluation/variation_calc2/toAvoid_DividedBy1 ==
  in_original : Inport
  Add3 : Sum
  Constant : Constant  Value=1e-10
  If : If  IfExpression=u1 == 0
  If Action Subsystem : Subsystem  TreatAsAtomicUnit=on
  If Action Subsystem1 : Subsystem  TreatAsAtomicUnit=on
  Merge : Merge
  in_processed : Outport
  wires:
  Merge/1 -> in_processed/1
  If/1 -> If Action Subsystem/Action
  If Action Subsystem1/1(Out1) -> Merge/2
  If/2 -> If Action Subsystem1/Action
  Constant/1 -> Add3/2
  If Action Subsystem/1(Out1) -> Merge/1
  Add3/1 -> If Action Subsystem1/1(In1)
  in_original/1 -> If/1, If Action Subsystem/1(In1), Add3/1

== system RLS_ADRC_2nd_order_Kang/learning_process_evaluation/variation_calc3/1st_order_LP_FIlter1 ==
  u : Inport
  T_sample : Inport  Port=2
  Add : Sum  Inputs=+-
  Add1 : Sum
  Delay : Delay  DelayLength=1
  Divide : Product  Inputs=*/
  Product2 : Product
  "tau_LPF " : Constant
  output : Outport
  wires:
  Add/1 -> Product2/2
  u/1 -> Add/1
  Add1/1 -> Delay/1, output/1
  T_sample/1 -> Product2/1
  Product2/1 -> Divide/1
  Delay/1 -> Add/2, Add1/2
  Divide/1 -> Add1/1
  "tau_LPF "/1 -> Divide/2

== system RLS_ADRC_2nd_order_Kang/learning_process_evaluation/variation_calc3/toAvoid_DividedBy0 ==
  in_original : Inport
  Add3 : Sum
  Constant : Constant  Value=1e-10
  If : If  IfExpression=u1 == 0
  If Action Subsystem : Subsystem  TreatAsAtomicUnit=on
  If Action Subsystem1 : Subsystem  TreatAsAtomicUnit=on
  Merge : Merge
  in_processed : Outport
  wires:
  in_original/1 -> Add3/1, If Action Subsystem/1(In1), If/1
  Add3/1 -> If Action Subsystem1/1(In1)
  If Action Subsystem/1(Out1) -> Merge/1
  Constant/1 -> Add3/2
  If/2 -> If Action Subsystem1/Action
  If Action Subsystem1/1(Out1) -> Merge/2
  If/1 -> If Action Subsystem/Action
  Merge/1 -> in_processed/1

== system RLS_ADRC_2nd_order_Kang/learning_process_evaluation/variation_calc4/1st_order_LP_FIlter1 ==
  u : Inport
  T_sample : Inport  Port=2
  Add : Sum  Inputs=+-
  Add1 : Sum
  Delay : Delay  DelayLength=1
  Divide : Product  Inputs=*/
  Product2 : Product
  "tau_LPF " : Constant
  output : Outport
  wires:
  "tau_LPF "/1 -> Divide/2
  Divide/1 -> Add1/1
  Delay/1 -> Add1/2, Add/2
  Product2/1 -> Divide/1
  T_sample/1 -> Product2/1
  Add1/1 -> output/1, Delay/1
  u/1 -> Add/1
  Add/1 -> Product2/2

== system RLS_ADRC_2nd_order_Kang/learning_process_evaluation/variation_calc4/toAvoid_DividedBy0 ==
  in_original : Inport
  Add3 : Sum
  Constant : Constant  Value=1e-10
  If : If  IfExpression=u1 == 0
  If Action Subsystem : Subsystem  TreatAsAtomicUnit=on
  If Action Subsystem1 : Subsystem  TreatAsAtomicUnit=on
  Merge : Merge
  in_processed : Outport
  wires:
  Merge/1 -> in_processed/1
  If/1 -> If Action Subsystem/Action
  If Action Subsystem1/1(Out1) -> Merge/2
  If/2 -> If Action Subsystem1/Action
  Constant/1 -> Add3/2
  If Action Subsystem/1(Out1) -> Merge/1
  Add3/1 -> If Action Subsystem1/1(In1)
  in_original/1 -> If/1, If Action Subsystem/1(In1), Add3/1

== system RLS_ADRC_2nd_order_Kang/learning_process_evaluation/variation_calc1/toAvoid_DividedBy0/If Action Subsystem ==
  In1 : Inport
  Action Port : ActionPort  ActionPortLabel=if(u1 == 0)
  Out1 : Outport
  wires:
  In1/1 -> Out1/1

== system RLS_ADRC_2nd_order_Kang/learning_process_evaluation/variation_calc1/toAvoid_DividedBy0/If Action Subsystem1 ==
  In1 : Inport
  Action Port : ActionPort  ActionPortLabel=else
  Out1 : Outport
  wires:
  In1/1 -> Out1/1

== system RLS_ADRC_2nd_order_Kang/learning_process_evaluation/variation_calc2/toAvoid_DividedBy0/If Action Subsystem ==
  In1 : Inport
  Action Port : ActionPort  ActionPortLabel=if(u1 < 1e-1 | u1>-1e-1)
  Out1 : Outport
  wires:
  In1/1 -> Out1/1

== system RLS_ADRC_2nd_order_Kang/learning_process_evaluation/variation_calc2/toAvoid_DividedBy0/If Action Subsystem1 ==
  in_original : Inport
  Action Port : ActionPort  ActionPortLabel=else
  Out1 : Outport
  wires:
  in_original/1 -> Out1/1

== system RLS_ADRC_2nd_order_Kang/learning_process_evaluation/variation_calc2/toAvoid_DividedBy1/If Action Subsystem ==
  In1 : Inport
  Action Port : ActionPort  ActionPortLabel=if(u1 == 0)
  Out1 : Outport
  wires:
  In1/1 -> Out1/1

== system RLS_ADRC_2nd_order_Kang/learning_process_evaluation/variation_calc2/toAvoid_DividedBy1/If Action Subsystem1 ==
  In1 : Inport
  Action Port : ActionPort  ActionPortLabel=else
  Out1 : Outport
  wires:
  In1/1 -> Out1/1

== system RLS_ADRC_2nd_order_Kang/learning_process_evaluation/variation_calc3/toAvoid_DividedBy0/If Action Subsystem ==
  In1 : Inport
  Action Port : ActionPort  ActionPortLabel=if(u1 == 0)
  Out1 : Outport
  wires:
  In1/1 -> Out1/1

== system RLS_ADRC_2nd_order_Kang/learning_process_evaluation/variation_calc3/toAvoid_DividedBy0/If Action Subsystem1 ==
  In1 : Inport
  Action Port : ActionPort  ActionPortLabel=else
  Out1 : Outport
  wires:
  In1/1 -> Out1/1

== system RLS_ADRC_2nd_order_Kang/learning_process_evaluation/variation_calc4/toAvoid_DividedBy0/If Action Subsystem ==
  In1 : Inport
  Action Port : ActionPort  ActionPortLabel=if(u1 == 0)
  Out1 : Outport
  wires:
  In1/1 -> Out1/1

== system RLS_ADRC_2nd_order_Kang/learning_process_evaluation/variation_calc4/toAvoid_DividedBy0/If Action Subsystem1 ==
  In1 : Inport
  Action Port : ActionPort  ActionPortLabel=else
  Out1 : Outport
  wires:
  In1/1 -> Out1/1

== matlab function RLS_ADRC_2nd_order_Kang/RLS with forgetting_factor ==
  data: K_k output; Lamb input; Phi_k input; Y_k input; Theta_k_1 input; Theta_k output; P_k output; P_k_1 input
function [K_k,Theta_k,P_k] = fcn(Lamb,Phi_k,Y_k,Theta_k_1,P_k_1)
%#codegen
%Kang Song
% 遗忘因子用于协方差更新；控制器采用新参数还要通过外层切换判据。
K_k=P_k_1*Phi_k/(Lamb+Phi_k'*P_k_1*Phi_k);
P_k=1./Lamb.*(eye(4,4)-K_k*Phi_k')*P_k_1;
Theta_k=Theta_k_1+K_k*(Y_k-Phi_k'*Theta_k_1);
